simulink model "test1"  (R2025b)
settings: Solver=FixedStepAuto  StartTime=0.0  StopTime=inf  FixedStep=0.01  RelTol=1e-3
model workspace (MAT data in the model file):
  SL_ROS_VariableLengthArrays_MaxSizes.CommonInfo.ArrayTruncateAction = 'EmitWarning'
  SL_ROS_VariableLengthArrays_MaxSizes.MsgTypeMap = containers.Map
  SL_ROS_VariableLengthArrays_MaxSizes.MsgTypeMap.serialization.keys = {'std_msgs/Float64MultiArray'}
  SL_ROS_VariableLengthArrays_MaxSizes.MsgTypeMap.serialization.values{1}.PropertyName = 'data'
  SL_ROS_VariableLengthArrays_MaxSizes.MsgTypeMap.serialization.values{1}.DataType = 'double'
  SL_ROS_VariableLengthArrays_MaxSizes.MsgTypeMap.serialization.values{1}.MaxLength = 4
  SL_ROS_VariableLengthArrays_MaxSizes.MsgTypeMap.serialization.uniformity = 0
  SL_ROS_VariableLengthArrays_MaxSizes.MsgTypeMap.serialization.keyType = 'char'
  SL_ROS_VariableLengthArrays_MaxSizes.MsgTypeMap.serialization.valueType = 'any'
values from neighbouring files (symbols this model uses):
  Ixx = 0.035    [AttitudeControl.m]    (also in quadrotor_dynamics.m = in4(4,:))
  Iyy = 0.07    [AttitudeControl.m]    (also in quadrotor_dynamics.m = in4(5,:))
  Izz = 0.098    [AttitudeControl.m]    (also in quadrotor_dynamics.m = in4(6,:))
  par = [m; g; beta; Ixx; Iyy; Izz; k; b; l]    [AttitudeControl.m]
undefined symbols (not defined in the file or in its folder): data, data_SL_Info, Kp, Kr, Kt
libraries: ros2lib x7, simulink x4, robotcorelib x2
settings Model: Creator=leo  LastModifiedBy=leo

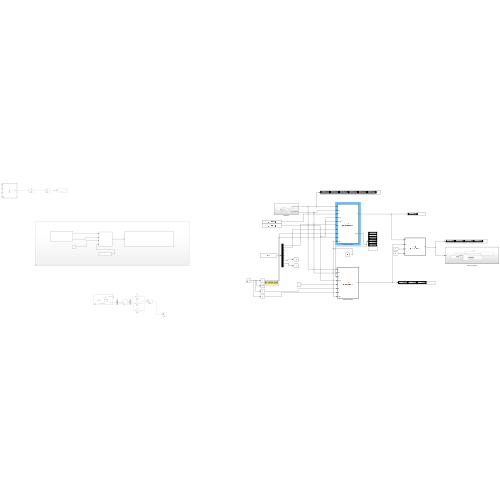
[thumbnail: Simulink's stored preview of the top-level diagram]
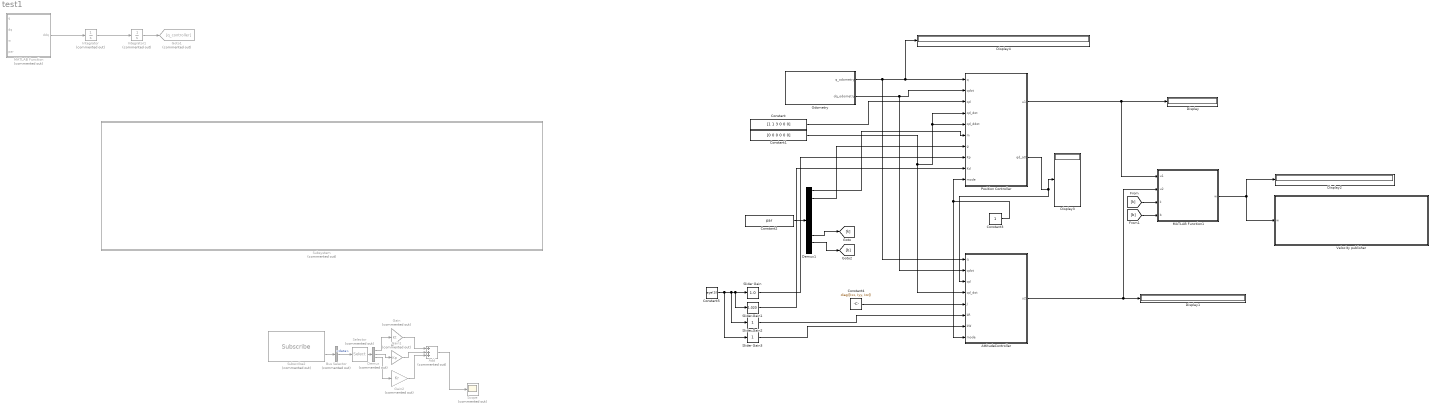
== system test1 ==
  Add : Sum  Commented=on  Inputs=+++
  AttitudeController : MATLAB Function  TreatAsAtomicUnit=on
  Bus Selector : BusSelector  Commented=on  OutputSignals=data
  Constant : Constant  Value=[1 1 3 0 0 0]
  Constant1 : Constant  Value=[0 0 0 0 0 0]
  Constant2 : Constant  Value=par
  Constant3 : Constant
  Constant4 : Constant  Value=diag([Ixx, Iyy, Izz])
  Constant5 : Constant  Value=eye(3)
  Demux : Demux  Commented=on  Outputs=3
  Demux1 : Demux  Outputs=9
  Display{,1..4} (5 alike) : Display
  Gain : Gain  Commented=on  Gain=Kt
  Gain1 : Gain  Commented=on  Gain=Kp
  Gain2 : Gain  Commented=on  Gain=Kr
  Goto1 : Goto  Commented=on  GotoTag=q_controller
  Integrator : Integrator  Commented=on  InitialCondition=zeros(6,1)
  Integrator1 : Integrator  Commented=on  InitialCondition=zeros(6,1)
  MATLAB Function : MATLAB Function  Commented=on  TreatAsAtomicUnit=on
  MATLAB Function1 : MATLAB Function  TreatAsAtomicUnit=on
  Odometry : Subsystem
  Position Controller : MATLAB Function  TreatAsAtomicUnit=on
  Scope : Scope  Commented=on
      settings: ActiveDisplayYMinimum=-420.549542851473  ActiveDisplayYMaximum=841.27315392614639
  Selector : Selector  Commented=on  InputPortWidth=128  IndexOptions=Index vector (dialog)  Indices=[1 2 3]  OutputSizes=1
  Slider Gain : simulink/Math Operations/Slider Gain  gain=1.0  low=0  high=100
  Slider Gain1 : simulink/Math Operations/Slider Gain  gain=1.020  low=0  high=2
  Slider Gain2 : simulink/Math Operations/Slider Gain  gain=1  low=0  high=2
  Slider Gain3 : simulink/Math Operations/Slider Gain  gain=1  low=0  high=2
  Subscribe2 : ros2lib/Subscribe  Commented=on  topicSource=Select from ROS network  topic=/Comandi  messageType=std_msgs/Float64MultiArray  sampleTime=-1  QOSHistory=Keep last  QOSDepth=10  QOSReliability=Reliable  QOSDurability=Volatile  QOSDeadline=Inf  QOSLifespan=Inf  QOSLiveliness=Automatic  QOSLeaseDuration=Inf  QOSAvoidROSNamespaceConventions=off
  Subsystem : Subsystem  Commented=on
  Velocity publisher : Subsystem
  wires:
  Gain/1 -> Add/1
  Gain1/1 -> Add/2
  Gain2/1 -> Add/3
  Add/1 -> Scope/1
  Subscribe2/2 -> Bus Selector/1
  Bus Selector/1 -> Selector/1  "<data>"
  Selector/1 -> Demux/1
  Demux/1 -> Gain/1
  Demux/2 -> Gain1/1
  Demux/3 -> Gain2/1
  MATLAB Function/1(ddq) -> Integrator/1
  Integrator/1 -> Integrator1/1
  Integrator1/1 -> Goto1/1
  Odometry/1(q_odometry) -> AttitudeController/1(q), Display4/1, Position Controller/1(q)
  Odometry/2(dq_odometry) -> AttitudeController/2(qdot), Position Controller/2(qdot)
  Constant/1 -> Position Controller/3(qd)
  Constant1/1 -> AttitudeController/4(qd_dot), Position Controller/5(qd_ddot), Position Controller/4(qd_dot)
  Constant2/1 -> Demux1/1
  Demux1/1 -> Position Controller/6(m)
  Demux1/2 -> Position Controller/7(g)
  Constant3/1 -> Position Controller/10(mode), AttitudeController/8(mode)
  Slider Gain/1 -> Position Controller/8(Kp)
  Slider Gain1/1 -> Position Controller/9(Kd)
  Slider Gain2/1 -> AttitudeController/6(kR)
  Slider Gain3/1 -> AttitudeController/7(kW)
  Position Controller/1(u1) -> MATLAB Function1/1(u1), Display/1
  AttitudeController/1(u2) -> MATLAB Function1/2(u2), Display1/1
  Constant4/1 -> AttitudeController/5(J)
  Demux1/7 -> [k]
  Demux1/8 -> [b]
  [k] -> MATLAB Function1/3(k)
  [b] -> MATLAB Function1/4(b)
  MATLAB Function1/1(w) -> Velocity publisher/1(w), Display2/1
  Position Controller/2(qd_att) -> AttitudeController/3(qd), Display3/1
  Constant5/1 -> Slider Gain3/1, Slider Gain2/1, Slider Gain1/1, Slider Gain/1

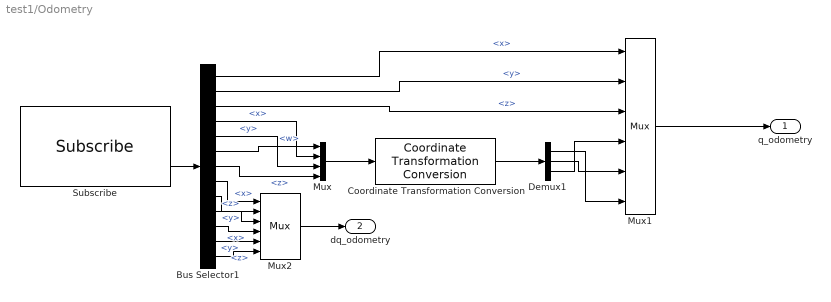
== system test1/Odometry ==
  Bus Selector1 : BusSelector  OutputSignals=pose.pose.position.x,pose.pose.position.y,pose.pose.position.z,pose.pose.orientation.x,pose.pose.orientation.y,pose.pose.orientation.w,pose.pose.orientation.z,twist.twist.linear.x,twist.twist.linear.y,twist.twist.linear.z,twist.twist.angular.x,twist.twist.angular.y,twist.twist.angular.z
  Coordinate Transformation Conversion : robotcorelib/Coordinate Transformation Conversion  InputRepresentation=Quaternion  InputEulerSequence=ZYX  ShowTrVecInputPort=on  OutputRepresentation=Euler Angles  OutputEulerSequence=ZYX  ShowTrVecOutputPort=on  SimulateUsing=Interpreted execution
      settings: LibrarySourceBlock=roslib/Utilities/Coordinate Transformation Conversion
  Demux1 : Demux  Outputs=3
  Mux : Mux
  Mux1 : Mux  Inputs=6
  Mux2 : Mux  Inputs=6
  Subscribe : ros2lib/Subscribe  topicSource=Select from ROS network  topic=/x3/odometry  messageType=nav_msgs/Odometry  sampleTime=-1  QOSHistory=Keep last  QOSDepth=10  QOSReliability=Reliable  QOSDurability=Volatile  QOSDeadline=Inf  QOSLifespan=Inf  QOSLiveliness=Automatic  QOSLeaseDuration=Inf  QOSAvoidROSNamespaceConventions=off
  q_odometry : Outport  VectorParamsAs1DForOutWhenUnconnected=off
  dq_odometry : Outport  Port=2  VectorParamsAs1DForOutWhenUnconnected=off
  wires:
  Mux/1 -> Coordinate Transformation Conversion/1
  Mux1/1 -> q_odometry/1
  Bus Selector1/13 -> Mux2/6  "<z>"
  Subscribe/2 -> Bus Selector1/1
  Demux1/2 -> Mux1/5
  Bus Selector1/9 -> Mux2/2  "<y>"
  Bus Selector1/3 -> Mux1/3  "<z>"
  Bus Selector1/7 -> Mux/4  "<z>"
  Bus Selector1/11 -> Mux2/4  "<x>"
  Bus Selector1/4 -> Mux/2  "<x>"
  Bus Selector1/12 -> Mux2/5  "<y>"
  Bus Selector1/2 -> Mux1/2  "<y>"
  Bus Selector1/8 -> Mux2/1  "<x>"
  Demux1/3 -> Mux1/4
  Bus Selector1/10 -> Mux2/3  "<z>"
  Bus Selector1/5 -> Mux/3  "<y>"
  Bus Selector1/6 -> Mux/1  "<w>"
  Mux2/1 -> dq_odometry/1
  Demux1/1 -> Mux1/6
  Coordinate Transformation Conversion/1 -> Demux1/1
  Bus Selector1/1 -> Mux1/1  "<x>"

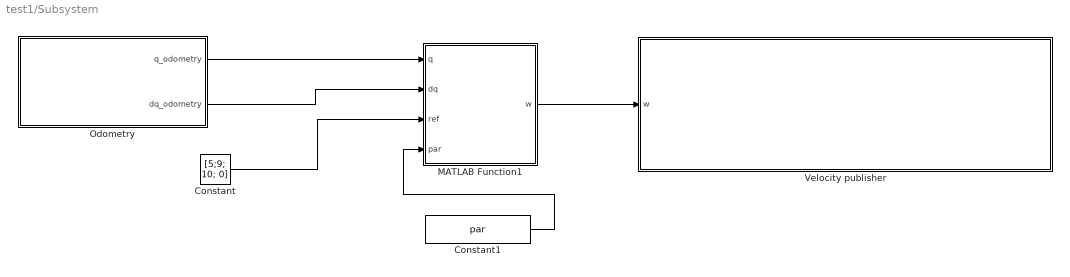
== system test1/Subsystem ==
  Constant : Constant  Value=[5;9; 10; 0]
  Constant1 : Constant  Value=par
  MATLAB Function1 : MATLAB Function  TreatAsAtomicUnit=on
  Odometry : Subsystem
  Velocity publisher : Subsystem
  wires:
  Constant/1 -> MATLAB Function1/3(ref)
  Odometry/1(q_odometry) -> MATLAB Function1/1(q)
  Odometry/2(dq_odometry) -> MATLAB Function1/2(dq)
  MATLAB Function1/1(w) -> Velocity publisher/1(w)
  Constant1/1 -> MATLAB Function1/4(par)

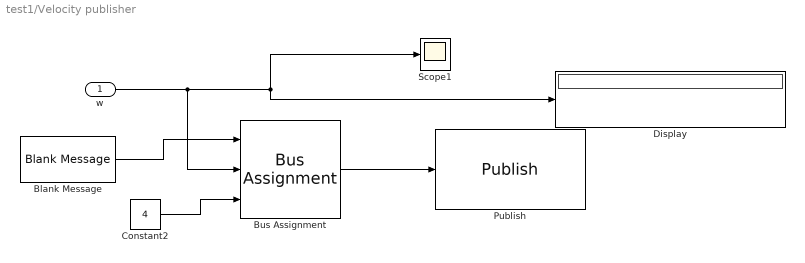
== system test1/Velocity publisher ==
  w : Inport
  Blank Message : ros2lib/Blank Message  messageClass=Message  entityType=std_msgs/Float64MultiArray  messageType=std_msgs/Float64MultiArray  SampleTime=inf
  Bus Assignment : BusAssignment  AssignedSignals=data,data_SL_Info.CurrentLength
  Constant2 : Constant  Value=4  OutDataTypeStr=uint32
  Display : Display
  Publish : ros2lib/Publish  topicSource=Select from ROS network  topic=/controllore/motor_speed  messageType=std_msgs/Float64MultiArray  QOSHistory=Keep last  QOSDepth=10  QOSReliability=Reliable  QOSDurability=Volatile  QOSDeadline=Inf  QOSLifespan=Inf  QOSLiveliness=Automatic  QOSLeaseDuration=Inf  QOSAvoidROSNamespaceConventions=off
  Scope1 : Scope
      settings: ActiveDisplayYMinimum=-144.32012748750208  ActiveDisplayYMaximum=986.44700405554
  wires:
  Constant2/1 -> Bus Assignment/3
  w/1 -> Bus Assignment/2, Scope1/1, Display/1
  Bus Assignment/1 -> Publish/1
  Blank Message/1 -> Bus Assignment/1

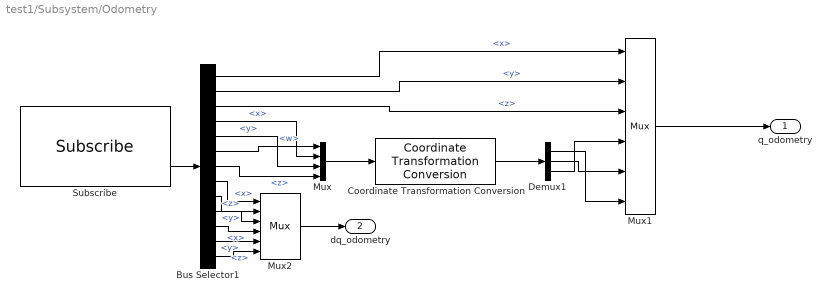
== system test1/Subsystem/Odometry ==
  Bus Selector1 : BusSelector  OutputSignals=pose.pose.position.x,pose.pose.position.y,pose.pose.position.z,pose.pose.orientation.x,pose.pose.orientation.y,pose.pose.orientation.w,pose.pose.orientation.z,twist.twist.linear.x,twist.twist.linear.y,twist.twist.linear.z,twist.twist.angular.x,twist.twist.angular.y,twist.twist.angular.z
  Coordinate Transformation Conversion : robotcorelib/Coordinate Transformation Conversion  InputRepresentation=Quaternion  InputEulerSequence=ZYX  ShowTrVecInputPort=on  OutputRepresentation=Euler Angles  OutputEulerSequence=ZYX  ShowTrVecOutputPort=on  SimulateUsing=Interpreted execution
      settings: LibrarySourceBlock=roslib/Utilities/Coordinate Transformation Conversion
  Demux1 : Demux  Outputs=3
  Mux : Mux
  Mux1 : Mux  Inputs=6
  Mux2 : Mux  Inputs=6
  Subscribe : ros2lib/Subscribe  topicSource=Select from ROS network  topic=/x3/odometry  messageType=nav_msgs/Odometry  sampleTime=-1  QOSHistory=Keep last  QOSDepth=10  QOSReliability=Reliable  QOSDurability=Volatile  QOSDeadline=Inf  QOSLifespan=Inf  QOSLiveliness=Automatic  QOSLeaseDuration=Inf  QOSAvoidROSNamespaceConventions=off
  q_odometry : Outport  VectorParamsAs1DForOutWhenUnconnected=off
  dq_odometry : Outport  Port=2  VectorParamsAs1DForOutWhenUnconnected=off
  wires:
  Mux/1 -> Coordinate Transformation Conversion/1
  Mux1/1 -> q_odometry/1
  Bus Selector1/13 -> Mux2/6  "<z>"
  Subscribe/2 -> Bus Selector1/1
  Demux1/2 -> Mux1/5
  Bus Selector1/9 -> Mux2/2  "<y>"
  Bus Selector1/3 -> Mux1/3  "<z>"
  Bus Selector1/7 -> Mux/4  "<z>"
  Bus Selector1/11 -> Mux2/4  "<x>"
  Bus Selector1/4 -> Mux/2  "<x>"
  Bus Selector1/12 -> Mux2/5  "<y>"
  Bus Selector1/2 -> Mux1/2  "<y>"
  Bus Selector1/8 -> Mux2/1  "<x>"
  Demux1/3 -> Mux1/4
  Bus Selector1/10 -> Mux2/3  "<z>"
  Bus Selector1/5 -> Mux/3  "<y>"
  Bus Selector1/6 -> Mux/1  "<w>"
  Mux2/1 -> dq_odometry/1
  Demux1/1 -> Mux1/6
  Coordinate Transformation Conversion/1 -> Demux1/1
  Bus Selector1/1 -> Mux1/1  "<x>"

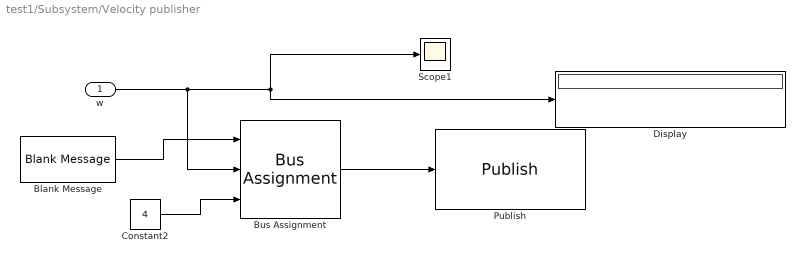
== system test1/Subsystem/Velocity publisher ==
  w : Inport
  Blank Message : ros2lib/Blank Message  messageClass=Message  entityType=std_msgs/Float64MultiArray  messageType=std_msgs/Float64MultiArray  SampleTime=inf
  Bus Assignment : BusAssignment  AssignedSignals=data,data_SL_Info.CurrentLength
  Constant2 : Constant  Value=4  OutDataTypeStr=uint32
  Display : Display
  Publish : ros2lib/Publish  topicSource=Select from ROS network  topic=/controllore/motor_speed  messageType=std_msgs/Float64MultiArray  QOSHistory=Keep last  QOSDepth=10  QOSReliability=Reliable  QOSDurability=Volatile  QOSDeadline=Inf  QOSLifespan=Inf  QOSLiveliness=Automatic  QOSLeaseDuration=Inf  QOSAvoidROSNamespaceConventions=off
  Scope1 : Scope
      settings: ActiveDisplayYMinimum=-144.32012748750208  ActiveDisplayYMaximum=986.44700405554
  wires:
  Constant2/1 -> Bus Assignment/3
  w/1 -> Bus Assignment/2, Scope1/1, Display/1
  Bus Assignment/1 -> Publish/1
  Blank Message/1 -> Bus Assignment/1

== matlab function test1/Subsystem/MATLAB Function1 ==
  data: q input; w output; dq input; ref input; par input
function w = ctrl(q, dq, ref, par)
m   = par(1); g   = par(2); 
Ixx = par(4); Iyy = par(5); Izz = par(6);
k   = par(7); b   = par(8);

Kp_p = 2.0;  Kd_p = 2.2;
Kp_a = 22.0; Kd_a = 6.0;

% 1. Anello esterno: posizione [x, y, z] in terna Gazebo (X avanti, Y sinistra, Z alto)
a  = Kp_p * (ref(1:3) - q(1:3)) - Kd_p * dq(1:3);
tz = q(6);

cos_tilt = max(cos(q(4)) * cos(q(5)), 0.5);
T = m * (g + a(3)) / cos_tilt;

txd = max(min(( a(1)*sin(tz) - a(2)*cos(tz)) / g, 0.35), -0.35);
tyd = max(min(( a(1)*cos(tz) + a(2)*sin(tz)) / g, 0.35), -0.35);
tzd = ref(4);

% 2. Anello interno: assetto
e    = [txd; tyd; tzd] - q(4:6);
e(3) = atan2(sin(e(3)), cos(e(3)));
tau  = diag([Ixx, Iyy, Izz]) * (Kp_a * e - Kd_a * dq(4:6));

% 3. Mixer inverso allineato a Gazebo (X avanti, Y sinistra, Z alto)
% Rotor 0: (+0.13, -0.22) CCW | Rotor 1: (-0.13, +0.20) CCW
% Rotor 2: (+0.13, +0.22) CW  | Rotor 3: (-0.13, -0.20) CW
A = [    k,        k,        k,        k;
      -0.22*k,   0.20*k,   0.22*k,  -0.20*k;   % Roll  (tau_x: motori dx vs sx)
      -0.13*k,   0.13*k,  -0.13*k,   0.13*k;   % Pitch (tau_y: motori avanti vs dietro)
        -b,       -b,        b,        b ];    % Yaw   (tau_z: CCW vs CW)

w2 = A \ [T; tau];
w  = min(sqrt(max(w2, 0)), 800);
end

== matlab function test1/MATLAB Function ==
  data: q input; ddq output; dq input; w input; par input
function ddq = f(q, dq, w, par)
    ddq = quadrotor_dynamics(q, dq, w, par);
end

== matlab function test1/AttitudeController ==
  data: q input; u2 output; qdot input; qd input; qd_dot input; J input; kR input; kW input; mode input
function u2 = attitudeController(q, qdot, qd, qd_dot, J, kR, kW, mode)
%ATTITUDECONTROLLER  Controllo di assetto su SO(3) per MATLAB Function block.
%
%   Mahony, Kumar, Corke, "Multirotor Aerial Vehicles", IEEE RAM 2012,
%   eq. (24)-(27). L'unica uscita e' u2 (momenti); u1 viene dal controllo
%   di traiettoria. La legge e' su SO(3) e non dipende dagli angoli:
%   gli angoli servono solo per costruire R e Rd.
%
%   CONVENZIONE
%     RPY Z-Y-X:  R = Rz(yaw)*Ry(pitch)*Rx(roll) = eul2rotm([yaw pitch roll],'ZYX')
%     R = ^A R_B  (v_A = R*v_B)
%
%   INGRESSI  (coordinate generalizzate, scomposte all'interno)
%     q       6x1  [x; y; z; roll; pitch; yaw]          letto
%     qdot    6x1  [dx; dy; dz; droll; dpitch; dyaw]    letto
%     qd      6x1  come q,    desiderato
%     qd_dot  6x1  come qdot, desiderato
%     J       3x3  matrice d'inerzia in {B} [kg m^2]
%     kR, kW  3x3  guadagni (definiti positivi, di solito diagonali)
%     mode    0 = PD lineare, eq. (26):  u2 = -kR*eR - kW*eW
%             1 = geometrico, eq. (27), valido anche per grandi rotazioni
%             (con Omega_d' = 0: i termini in Omega_d' si trascurano)
%
%   Se il tuo vettore q ha un ordine diverso, cambia solo i quattro
%   indici nella sezione "scomposizione" qui sotto.
%
%   USCITA
%     u2  3x1  momenti (tau_x, tau_y, tau_z) in {B} [N m]
%
%   GUADAGNI
%     mode 0: kR [N m/rad], kW [N m s/rad]  -> kR = J*wn^2,  kW = 2*J*wn
%     mode 1: J moltiplica i guadagni       -> kR = wn^2*I,  kW = 2*wn*I
%
%   SEGNO: con e_R^x = 1/2 (Rd'*R - R'*Rd), e_R e' "attuale - desiderato",
%   quindi la retroazione ha segno meno.

    % --- scomposizione: solo gli angoli e le loro derivate ---
    eul    = [q(6),      q(5),      q(4)];        % [yaw pitch roll]
    deul   = [qdot(6),   qdot(5),   qdot(4)];     % derivate degli angoli
    eulD   = [qd(6),     qd(5),     qd(4)];
    deulD  = [qd_dot(6), qd_dot(5), qd_dot(4)];

    % --- derivate degli angoli -> velocita' angolare del corpo in {B} ---
    Omega   = eulRate2omega(eul,  deul);
    Omega_d = eulRate2omega(eulD, deulD);

    % --- matrici di rotazione (funzione standard UAV Toolbox) ---
    R  = eul2rotm(eul,  'ZYX');
    Rd = eul2rotm(eulD, 'ZYX');

    % --- errore di assetto, eq. (24) ---
    eR = vee(0.5 * (Rd' * R - R' * Rd));

    if mode == 0
        % --- PD lineare, eq. (26) ---
        eW = Omega - Omega_d;
        u2 = -kR * eR - kW * eW;
    else
        % --- controllore geometrico, eq. (27), con dOmega_d = 0 ---
        RtRd = R' * Rd;
        eW   = Omega - RtRd * Omega_d;
        u2   = J * (-kR * eR - kW * eW) ...
             + cross(Omega, J * Omega) ...
             - J * (hat(Omega) * RtRd * Omega_d);
    end
end

function w = eulRate2omega(eul, deul)
%EULRATE2OMEGA  [dyaw dpitch droll] -> velocita' angolare (p,q,r) in {B}, Z-Y-X
    pitch = eul(2);  roll = eul(3);
    dyaw  = deul(1); dpitch = deul(2); droll = deul(3);
    w = [ droll - sin(pitch)*dyaw;
          cos(roll)*dpitch + sin(roll)*cos(pitch)*dyaw;
         -sin(roll)*dpitch + cos(roll)*cos(pitch)*dyaw ];
end

function S = hat(v)
%HAT  v -> v^x, tale che hat(v)*u = cross(v,u)
    S = [  0,   -v(3),  v(2);
          v(3),   0,   -v(1);
         -v(2),  v(1),   0 ];
end

function v = vee(S)
%VEE  inversa di hat
    v = [S(3,2); S(1,3); S(2,1)];
end

== matlab function test1/Position Controller ==
  data: q input; u1 output; qdot input; qd input; qd_dot input; qd_ddot input; m input; g input; Kp input; Kd input; mode input; qd_att output
function [u1, qd_att] = positionController(q, qdot, qd, qd_dot, qd_ddot, m, g, Kp, Kd, mode)
%POSITIONCONTROLLER  Controllo di traiettoria/posizione per MATLAB Function block.
%
%   Mahony, Kumar, Corke, "Multirotor Aerial Vehicles", IEEE RAM 2012,
%   eq. (28)-(31) e Fig. 5. Fornisce la spinta u1 e l'assetto desiderato
%   da passare a attitudeController (stesso formato di coordinate).
%
%   CONVENZIONE
%     {A} inerziale con z verso l'alto, RPY Z-Y-X:
%     R = Rz(yaw)*Ry(pitch)*Rx(roll)
%
%   INGRESSI  (coordinate generalizzate, scomposte all'interno)
%     q        6x1  [x; y; z; roll; pitch; yaw]          letto
%     qdot     6x1  [dx; dy; dz; droll; dpitch; dyaw]    letto
%     qd       6x1  come q,    desiderato (si usano x y z e yaw)
%     qd_dot   6x1  come qdot, desiderato (si usano dx dy dz)
%     qd_ddot  6x1  accelerazione desiderata (si usano ddx ddy ddz; zeros
%                   per regolazione a un punto fisso)
%     m        massa [kg]
%     g        accelerazione di gravita' [m/s^2]  (9.81)
%     Kp, Kd   3x3  guadagni di posizione e velocita' (diagonali, > 0)
%     mode     0 = lineare, eq. (29)-(30): u1 = m(g + acom_z), angoli da (30a,b)
%              1 = non lineare, eq. (31): u1 = m*b3'*(acom + g*a3),
%                  assetto desiderato dalla piattezza differenziale
%
%   USCITE
%     u1      spinta totale [N]
%     qd_att  6x1  [xd; yd; zd; roll*; pitch*; yaw*]  -> ingresso qd di
%             attitudeController (con qd_dot = zeros se non serve)
%
%   GUADAGNI: Kp = wn^2*eye(3), Kd = 2*wn*eye(3). L'anello di posizione deve
%   essere piu' lento di quello di assetto (es. wn = 2..3 rad/s contro ~10).

    % --- scomposizione: posizione, velocita' e angolo di imbardata ---
    xi     = q(1:3);        dxi    = qdot(1:3);
    xiD    = qd(1:3);       dxiD   = qd_dot(1:3);   ddxiD = qd_ddot(1:3);
    psiD   = qd(6);                                  % yaw desiderato

    a3 = [0; 0; 1];

    % --- accelerazione comandata: PD + feedforward ---
    acom = ddxiD + Kd * (dxiD - dxi) + Kp * (xiD - xi);

    if mode == 0
        % --- lineare, eq. (29) e (30a,b) ---
        u1     = m * (g + acom(3));
        phiD   = (acom(1) * sin(psiD) - acom(2) * cos(psiD)) / g;
        thetaD = (acom(1) * cos(psiD) + acom(2) * sin(psiD)) / g;
        yawD   = psiD;
    else
        % --- non lineare, eq. (31) ---
        phi   = q(4);
        theta = q(5);
        psi   = q(6);

        % R = Rz(psi) * Ry(theta) * Rx(phi)
        R  = [ cos(psi)*cos(theta),  cos(psi)*sin(theta)*sin(phi) - sin(psi)*cos(phi),  cos(psi)*sin(theta)*cos(phi) + sin(psi)*sin(phi);
               sin(psi)*cos(theta),  sin(psi)*sin(theta)*sin(phi) + cos(psi)*cos(phi),  sin(psi)*sin(theta)*cos(phi) - cos(psi)*sin(phi);
              -sin(theta),           cos(theta)*sin(phi),                                cos(theta)*cos(phi) ];
        b3 = R(:, 3);
        u1 = m * (b3' * (acom + g * a3));

        % assetto desiderato (piattezza differenziale):
        %   b3* ~ forza richiesta, b2* = b3* x e1 / |.|, b1* = b2* x b3*
        f   = acom + g * a3;
        b3d = f / norm(f);
        e1  = [cos(psiD); sin(psiD); 0];
        b2d = cross(b3d, e1);
        b2d = b2d / norm(b2d);
        b1d = cross(b2d, b3d);

        Rd     = [b1d, b2d, b3d];
        yawD   = atan2(Rd(2,1), Rd(1,1));
        thetaD = atan2(-Rd(3,1), hypot(Rd(1,1), Rd(2,1)));
        phiD   = atan2(Rd(3,2), Rd(3,3));
    end

    qd_att = [xiD; phiD; thetaD; yawD];
end

== matlab function test1/MATLAB Function1 ==
  data: u1 input; w output; u2 input; k input; b input
function w = MotorController(u1,u2,k,b)





A = [    k,        k,        k,        k;
      -0.22*k,   0.20*k,   0.22*k,  -0.20*k;   % Roll  (tau_x: motori dx vs sx)
      -0.13*k,   0.13*k,  -0.13*k,   0.13*k;   % Pitch (tau_y: motori avanti vs dietro)
        -b,       -b,        b,        b ]; 
w2 = A \ [u1; u2];
w  = min(sqrt(max(w2, 0)), 800);
